simulink subsystem "mission_manager_interface"  (R2026a)
settings: Solver=VariableStepAuto
undefined symbols (not defined in the file): S
libraries: ros2lib x3
PreSaveFcn:
  | defaultToFileBlockNames(bdroot);
settings Model: Creator=kjhaydon  LastModifiedBy=kjhaydon

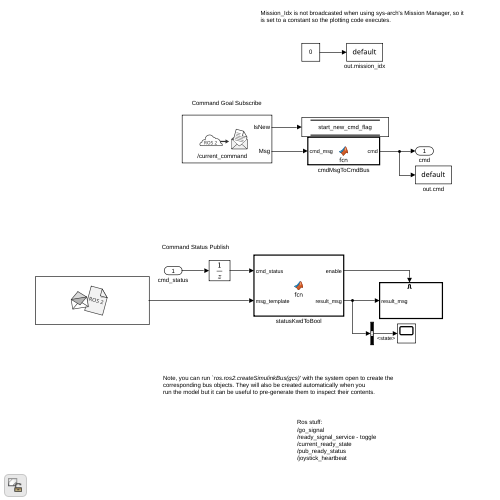
[thumbnail: Simulink's stored preview of the top-level diagram]
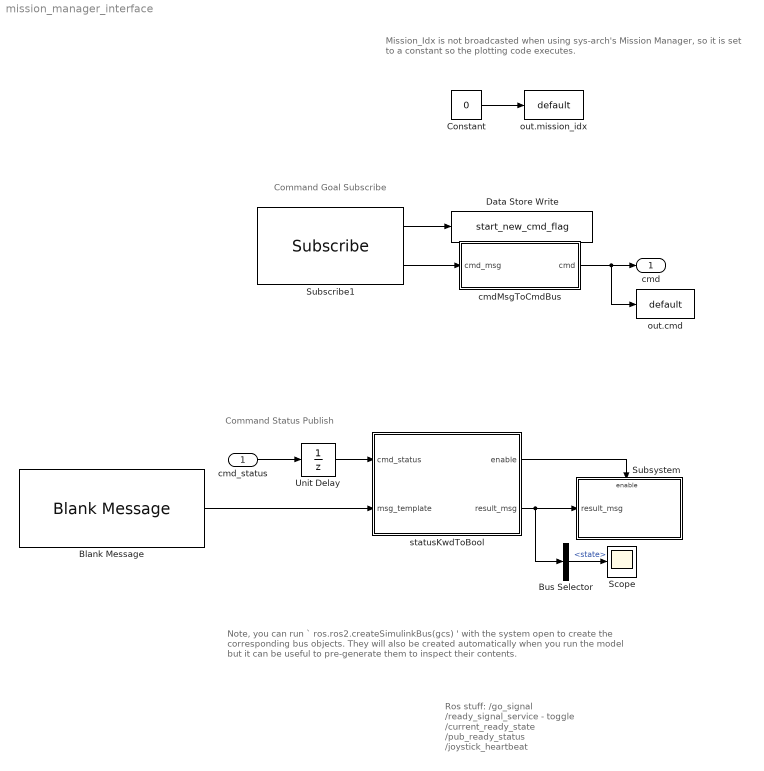
== system mission_manager_interface ==
  note: Ros stuff:
      | /go_signal
      | /ready_signal_service - toggle
      | /current_ready_state
      | /pub_ready_status
      | /joystick_heartbeat
  note: Note, you can run ` ros.ros2.createSimulinkBus(gcs) ' with the system open to create the
      | corresponding bus objects. They will also be created automatically when you
      | run the model but it can be useful to pre-generate them to inspect their contents.
  note: Command Status Publish
  note: Command Goal Subscribe
  note: Mission_Idx is not broadcasted when using sys-arch's Mission Manager, so it
      | is set to a constant so the plotting code executes.
  cmd_status : Inport  SampleTime=S.dt_control
  Blank Message : ros2lib/Blank Message  messageClass=Message  entityType=custom_interfaces/CommandResult  messageType=custom_interfaces/CommandResult  SampleTime=inf
  Bus Selector : BusSelector  OutputSignals=state
  Constant : Constant  Value=0
  Data Store Write : DataStoreWrite  DataStoreName=start_new_cmd_flag  SampleTime=S.dt_control  IndexOptions=Index vector (dialog)  Indices=1  OutputSizes=1
  Scope : Scope
      settings: ActiveDisplayYMinimum=-1  ActiveDisplayYMaximum=1  DataLoggingVariableName=ScopeData3
  Subscribe1 : ros2lib/Subscribe  topicSource=Specify your own  topic=/current_command  messageType=custom_interfaces/Command  sampleTime=-1  QOSHistory=Keep last  QOSDepth=10  QOSReliability=Reliable  QOSDurability=Volatile  QOSDeadline=Inf  QOSLifespan=Inf  QOSLiveliness=Automatic  QOSLeaseDuration=Inf  QOSAvoidROSNamespaceConventions=off
  Subsystem : Subsystem
  Unit Delay : UnitDelay  SampleTime=-1
  cmdMsgToCmdBus : MATLAB Function  TreatAsAtomicUnit=on
  out.cmd : ToFile  Filename=default  MatrixName=cmd  SaveFormat=Timeseries
  out.mission_idx : ToFile  Filename=default  MatrixName=mission_idx  SaveFormat=Timeseries
  statusKwdToBool : MATLAB Function  TreatAsAtomicUnit=on
  cmd : Outport  SampleTime=S.dt_control
  wires:
  cmd_status/1 -> Unit Delay/1
  statusKwdToBool/1(enable) -> Subsystem/Enable
  Unit Delay/1 -> statusKwdToBool/1(cmd_status)
  statusKwdToBool/2(result_msg) -> Subsystem/1(result_msg), Bus Selector/1
  Subscribe1/1 -> Data Store Write/1
  cmdMsgToCmdBus/1(cmd) -> out.cmd/1, cmd/1
  Subscribe1/2 -> cmdMsgToCmdBus/1(cmd_msg)
  Blank Message/1 -> statusKwdToBool/2(msg_template)
  Bus Selector/1 -> Scope/1  "<state>"
  Constant/1 -> out.mission_idx/1

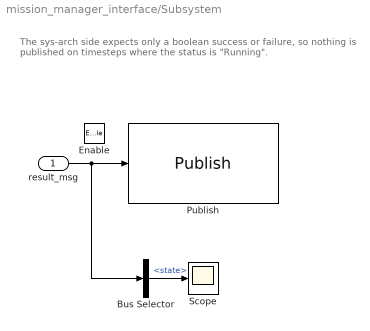
== system mission_manager_interface/Subsystem ==
  note: The sys-arch side expects only a boolean success or failure, so nothing
      | is published on timesteps where the status is "Running".
  result_msg : Inport
  Enable : EnablePort
  Bus Selector : BusSelector  OutputSignals=state
  Publish : ros2lib/Publish  topicSource=Specify your own  topic=/command_result  messageType=custom_interfaces/CommandResult  QOSHistory=Keep last  QOSDepth=10  QOSReliability=Reliable  QOSDurability=Volatile  QOSDeadline=Inf  QOSLifespan=Inf  QOSLiveliness=Automatic  QOSLeaseDuration=Inf  QOSAvoidROSNamespaceConventions=off
  Scope : Scope
      settings: DataLoggingVariableName=ScopeData2
  wires:
  Bus Selector/1 -> Scope/1  "<state>"
  result_msg/1 -> Publish/1, Bus Selector/1

== matlab function mission_manager_interface/cmdMsgToCmdBus ==
  data: cmd_msg input Bus: SL_Bus_custom_interfaces_Command; cmd output Bus: cmd_bus
function cmd = fcn(cmd_msg)

cmd = cmdMsgToCmdBus(cmd_msg);

end

== matlab function mission_manager_interface/statusKwdToBool ==
  data: enable output; cmd_status input; result_msg output Bus: SL_Bus_custom_interfaces_CommandResult; msg_template input Bus: SL_Bus_custom_interfaces_CommandResult
function [enable, result_msg]   = fcn(cmd_status, msg_template)

[enable, result_msg] = statusKwdToBool(cmd_status, msg_template);
